simulink model "Lab5_Team_13_ES3011_Simulink"  (R2024b)
settings: Solver=VariableStepAuto  StartTime=0.0  StopTime=120  RelTol=1e-3
values from neighbouring files (symbols this model uses):
  b = 3.5*10^(-6)    (= 3.5e-06)    [Lab5_Team_13_ES3011_B26.m]
  m = 1500    [Lab5_Team_13_ES3011_B26.m]
settings Model: Creator=aditi  LastModifiedBy=aditi

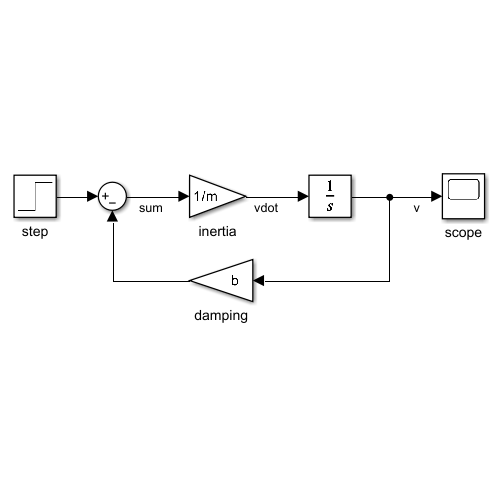
[thumbnail: Simulink's stored preview of the top-level diagram]
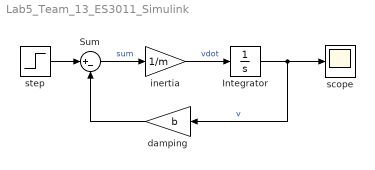
== system Lab5_Team_13_ES3011_Simulink ==
  Integrator : Integrator
  Sum : Sum  Inputs=|+-
  damping : Gain  Gain=b
  inertia : Gain  Gain=1/m
  scope : Scope
  step : Step  Time=0  After=u  SampleTime=0
  wires:
  inertia/1 -> Integrator/1  "vdot"
  Integrator/1 -> scope/1, damping/1  "v"
  Sum/1 -> inertia/1  "sum"
  damping/1 -> Sum/2
  step/1 -> Sum/1
